simulink model "Sistema_4_2024b"  (R2024b)
settings: Solver=ode15s  StartTime=0.0  StopTime=10  MaxStep=1E-2  RelTol=1e-3
libraries: fl_lib x14, nesl_utility x6, slpidlib x1
settings Model: LastModifiedBy=Ernesto
settings DataIOCC: SaveFormat=Array  SaveOutput=off  SignalLogging=off  DSMLogging=off  ReturnWorkspaceOutputs=off  TimeSaveName=t
settings DebuggingCC: AlgebraicLoopMsg=none  ArtificialAlgebraicLoopMsg=none  MaxConsecutiveZCsMsg=none
settings ModelReferenceCC: UpdateModelReferenceTargets=IfOutOfDate
settings RTWCC: GPUComputeCapability=7.5
settings ConfigComp: CovMetricSettings=de  CovBoundaryAbsTol=1.0e-5
settings SimscapeCC: SimscapeNominalValues="[{\"value\":\"1\",\"unit\":\"A\"},{\"value\":\"1\",\"unit\":\"bar\"},{\"value\":\"1\",\"unit\":\"cm^2\"},{\"value\":\"1\",\"unit\":\"cm^3/s\"},{\"value\":\"1\",\"unit\":\"kJ/kg\"},{\"value\":\"1\",\"unit\":\"kW\"},{\"value\":\"1\",\"unit\":\"l\"},{\"value\":\"1\",\"unit\":\"N\"},{\"value\":\"1\",\"unit\":\"N*m\"},{\"value\":\"1\",\"unit\":\"V\"},{\"value\":\"0.001\",\"unit\":\"Wb\"}]"  SimscapeLogType=all  SimscapeLogDataHistory=10000  SimscapeUseEnergyAccounting=off

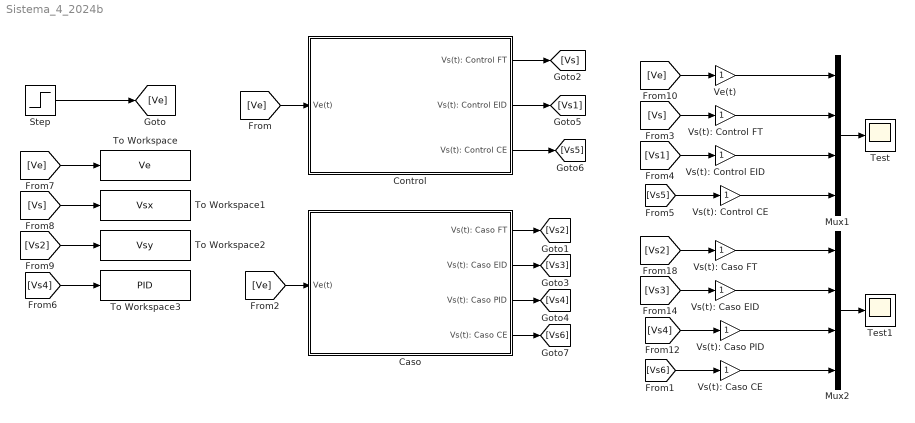
== system Sistema_4_2024b ==
  " Ve(t)" : Gain
  " Vs(t): Caso CE" : Gain
  " Vs(t): Caso EID" : Gain
  " Vs(t): Caso FT" : Gain
  " Vs(t): Caso PID" : Gain
  " Vs(t): Control CE" : Gain
  " Vs(t): Control EID" : Gain
  " Vs(t): Control FT" : Gain
  Caso : Subsystem
  Control : Subsystem
  Mux1 : Mux
  Mux2 : Mux
  Step : Step  Time=0  SampleTime=0
  Test : Scope
  Test1 : Scope
  To Workspace : ToWorkspace  VariableName=Ve  SampleTime=-1
  To Workspace1 : ToWorkspace  VariableName=Vsx  SampleTime=-1
  To Workspace2 : ToWorkspace  VariableName=Vsy  SampleTime=-1
  To Workspace3 : ToWorkspace  VariableName=PID  SampleTime=-1
  wires:
  [Ve] -> Control/1(Ve(t))
  Control/1(Vs(t): Control FT) -> [Vs]
  [Ve] -> Caso/1(Ve(t))
  Caso/1(Vs(t): Caso FT) -> [Vs2]
  Mux1/1 -> Test/1
  [Vs] -> " Vs(t): Control FT"/1
  [Vs1] -> " Vs(t): Control EID"/1
  Step/1 -> [Ve]
  Caso/2(Vs(t): Caso EID) -> [Vs3]
  [Ve] -> " Ve(t)"/1
  " Vs(t): Control FT"/1 -> Mux1/2
  " Ve(t)"/1 -> Mux1/1
  " Vs(t): Control EID"/1 -> Mux1/3
  Control/2(Vs(t): Control EID) -> [Vs1]
  [Ve] -> To Workspace/1
  [Vs] -> To Workspace1/1
  [Vs2] -> To Workspace2/1
  Caso/3(Vs(t): Caso PID) -> [Vs4]
  Control/3(Vs(t): Control CE) -> [Vs5]
  [Vs5] -> " Vs(t): Control CE"/1
  [Vs4] -> " Vs(t): Caso PID"/1
  [Vs3] -> " Vs(t): Caso EID"/1
  [Vs2] -> " Vs(t): Caso FT"/1
  Mux2/1 -> Test1/1
  " Vs(t): Control CE"/1 -> Mux1/4
  Caso/4(Vs(t): Caso CE) -> [Vs6]
  [Vs6] -> " Vs(t): Caso CE"/1
  " Vs(t): Caso FT"/1 -> Mux2/1
  " Vs(t): Caso EID"/1 -> Mux2/2
  " Vs(t): Caso PID"/1 -> Mux2/3
  " Vs(t): Caso CE"/1 -> Mux2/4
  [Vs4] -> To Workspace3/1

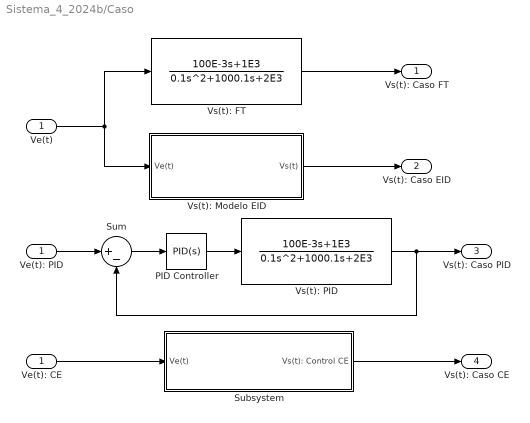
== system Sistema_4_2024b/Caso ==
  Ve(t) : Inport
  PID Controller : slpidlib/PID Controller  Controller=PID  Form=Parallel  TimeDomain=Continuous-time  UseExternalTs=off  SampleTime=-1  IntegratorMethod=Forward Euler  FilterMethod=Forward Euler  ControllerParametersSource=internal  P=13209.9564  I=32316525.9285  UseKiTs=off  D=0.18118  UseExternalDerivativeSource=off  N=521.395873847586  UseFilter=on  TunerSelectOption=Transfer Function Based (PID Tuner App)  InitialConditionSource=internal  InitialConditionForIntegrator=0  InitialConditionForFilter=0  DifferentiatorICPrevScaledInput=0  ExternalReset=none  TrackingMode=off  Kt=1  LimitOutput=off  SatLimitsSource=internal  UpperSaturationLimit=inf  LowerSaturationLimit=-inf  LinearizeAsGain=on  AntiWindupMode=none  Kb=1  LimitIntegrator=off  UpperIntegratorSaturationLimit=inf  LowerIntegratorSaturationLimit=-inf  POutMin=[]  POutMax=[]  IOutMin=[]  IOutMax=[]  DOutMin=[]  DOutMax=[]  NOutMin=[]  NOutMax=[]  SumOutMin=[]  SumOutMax=[]  SaturationOutMin=[]  SaturationOutMax=[]  PParamMin=[]  PParamMax=[]  IParamMin=[]  IParamMax=[]  DParamMin=[]  DParamMax=[]  NParamMin=[]  NParamMax=[]  KbParamMin=[]  KbParamMax=[]  KtParamMin=[]  KtParamMax=[]  KbOutMin=[]  KbOutMax=[]  KtOutMin=[]  KtOutMax=[]  IntegratorOutMin=[]  IntegratorOutMax=[]  FilterOutMin=[]  FilterOutMax=[]  SumI1OutMin=[]  SumI1OutMax=[]  SumI2OutMin=[]  SumI2OutMax=[]  SumI3OutMin=[]  SumI3OutMax=[]  SumI4OutMin=[]  SumI4OutMax=[]  SumDOutMin=[]  SumDOutMax=[]  DifferentiatorOutMin=[]  DifferentiatorOutMax=[]  FilterDiffOutCoefMin=[]  FilterDiffOutCoefMax=[]  ReciprocalOutMin=[]  ReciprocalOutMax=[]  SumDenOutMin=[]  SumDenOutMax=[]  SumNumOutMin=[]  SumNumOutMax=[]  DivideOutMin=[]  DivideOutMax=[]  UdiffTsProdOutMin=[]  UdiffTsProdOutMax=[]  NTsProdOutMin=[]  NTsProdOutMax=[]  UintegralTsProdOutMin=[]  UintegralTsProdOutMax=[]  UngainTsProdOutMin=[]  UngainTsProdOutMax=[]  ClampingZeroOutDataTypeStr=Inherit: Inherit via back propagation  ClampingZeroOutMin=[]  ClampingZeroOutMax=[]  FilterDenConstantOutDataTypeStr=Inherit: Inherit via back propagation  FilterDenConstantOutMin=[]  FilterDenConstantOutMax=[]  PCopyOutDataTypeStr=Inherit: Inherit via back propagation  PCopyOutMin=[]  PCopyOutMax=[]  NCopyOutDataTypeStr=Inherit: Inherit via back propagation  NCopyOutMin=[]  NCopyOutMax=[]  IntegratorContinuousStateAttributes=''  IntegratorStateMustResolveToSignalObject=off  IntegratorRTWStateStorageClass=Auto  FilterContinuousStateAttributes=''  FilterStateMustResolveToSignalObject=off  FilterRTWStateStorageClass=Auto  ParallelPVariant=InternalParameters  IdealPVariant=Disabled  IVariant=InternalParameters  DVariant=InternalParameters  IntegratorVariant=Continuous  SatVariant=Disabled  AWVariant=Passthrough  PCopyVariant=Disabled  TRVariant=Disabled  FdbkBlocksVariant=Forward  IdealPFdbkVariant=Disabled  SatFdbkVariant=Disabled  DerivativeFilterVariant=ContFilter  NVariant=InternalParameters  NCopyVariant=Disabled  FilterICVariant=InternalICsFilter  IntegratorICVariant=InternalICs  ExternalResetVariant=Disabled  TRSumVariant=Passthrough  SumFdbkVariant=Disabled  SumVariant=Sum_PID  TsampFilterVariant=InternalTs  TsampNgainVariant=Passthrough  TsampIntegralVariant=Disabled_SignalSpec  ExternalSaturationOutDataTypeStr=Inherit: Same as second input  DerivativeSourceVariant=ErrorSignal  PreIntVariant=InternalPreInt
  Subsystem : Subsystem
  Sum : Sum  Inputs=|+-
  Ve(t): CE : InportShadow
  Ve(t): PID : InportShadow
  Vs(t): FT : TransferFcn  Numerator=[100E-3, 1E3]  Denominator=[0.1, 1000.1, 2E3]
  Vs(t): Modelo EID : Subsystem
  Vs(t): PID : TransferFcn  Numerator=[100E-3, 1E3]  Denominator=[0.1, 1000.1, 2E3]
  Vs(t): Caso FT : Outport
  Vs(t): Caso EID : Outport  Port=2
  Vs(t): Caso PID : Outport  Port=3
  Vs(t): Caso CE : Outport  Port=4
  wires:
  Ve(t)/1 -> Vs(t): Modelo EID/1(Ve(t)), Vs(t): FT/1
  Vs(t): FT/1 -> Vs(t): Caso FT/1
  Vs(t): Modelo EID/1(Vs(t)) -> Vs(t): Caso EID/1
  PID Controller/1 -> Vs(t): PID/1
  Sum/1 -> PID Controller/1
  Ve(t): PID/1 -> Sum/1
  Vs(t): PID/1 -> Sum/2, Vs(t): Caso PID/1
  Ve(t): CE/1 -> Subsystem/1(Ve(t))
  Subsystem/1(Vs(t): Control CE) -> Vs(t): Caso CE/1

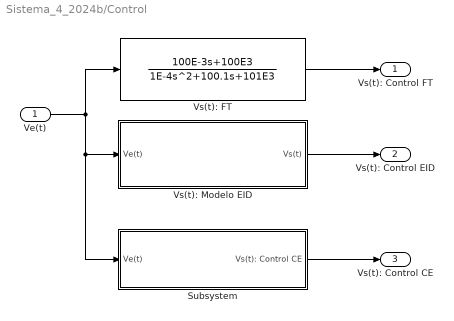
== system Sistema_4_2024b/Control ==
  Ve(t) : Inport
  Subsystem : Subsystem
  Vs(t): FT : TransferFcn  Numerator=[100E-3, 100E3]  Denominator=[1E-4, 100.1, 101E3]
  Vs(t): Modelo EID : Subsystem
  Vs(t): Control FT : Outport
  Vs(t): Control EID : Outport  Port=2
  Vs(t): Control CE : Outport  Port=3
  wires:
  Ve(t)/1 -> Subsystem/1(Ve(t)), Vs(t): Modelo EID/1(Ve(t)), Vs(t): FT/1
  Vs(t): FT/1 -> Vs(t): Control FT/1
  Vs(t): Modelo EID/1(Vs(t)) -> Vs(t): Control EID/1
  Subsystem/1(Vs(t): Control CE) -> Vs(t): Control CE/1

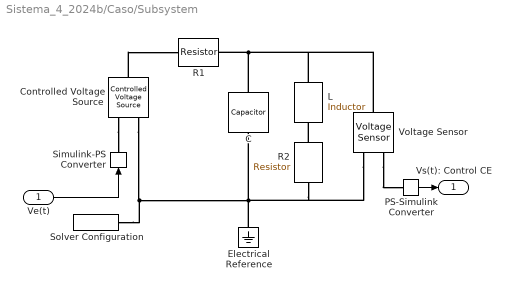
== system Sistema_4_2024b/Caso/Subsystem ==
  Ve(t) : Inport
  C : fl_lib/Electrical/Electrical Elements/Capacitor  c=1000 uF  r=1e-6 Ohm  g=0 1/Ohm  i_specify=off  i_priority=None  i=0 A  i_nominal_specify=off  i_nominal_value=1  i_nominal_unit=A  v_specify=off  v_priority=None  v=0 V  v_nominal_specify=off  v_nominal_value=1  v_nominal_unit=V  vc_specify=off  vc_priority=High  vc=0 V  vc_nominal_specify=off  vc_nominal_value=1  vc_nominal_unit=V
  Controlled Voltage Source : fl_lib/Electrical/Electrical Sources/Controlled Voltage Source
  Electrical Reference : fl_lib/Electrical/Electrical Elements/Electrical Reference
  L : fl_lib/Electrical/Electrical Elements/Inductor  l=100 mH  r=0 Ohm  g=1e-9 1/Ohm  i_specify=off  i_priority=None  i=0 A  i_nominal_specify=off  i_nominal_value=1  i_nominal_unit=A  v_specify=off  v_priority=None  v=0 V  v_nominal_specify=off  v_nominal_value=1  v_nominal_unit=V  i_L_specify=off  i_L_priority=High  i_L=0 A  i_L_nominal_specify=off  i_L_nominal_value=1  i_L_nominal_unit=A
  PS-Simulink Converter : nesl_utility/PS-Simulink Converter  PhysicalDomain=network_engine_domain  SubClassName=ps_output  LeftPortType=input  RightPortType=output  PseudoPeriodic=off  Frequencies=[]  VectorFormat=inherit  Unit=inherit  AffineConversion=off
  R1 : fl_lib/Electrical/Electrical Elements/Resistor  R=1 kOhm  i_specify=off  i_priority=None  i=0 A  i_nominal_specify=off  i_nominal_value=1  i_nominal_unit=A  v_specify=off  v_priority=None  v=0 V  v_nominal_specify=off  v_nominal_value=1  v_nominal_unit=V
  R2 : fl_lib/Electrical/Electrical Elements/Resistor  R=1 kOhm  i_specify=off  i_priority=None  i=0 A  i_nominal_specify=off  i_nominal_value=1  i_nominal_unit=A  v_specify=off  v_priority=None  v=0 V  v_nominal_specify=off  v_nominal_value=1  v_nominal_unit=V
  Simulink-PS Converter : nesl_utility/Simulink-PS Converter  PhysicalDomain=network_engine_domain  SubClassName=ps_input  LeftPortType=input  RightPortType=output  PseudoPeriodic=off  Frequencies=[]  NoiseDistribution=none  NoiseParameters=[]  Unit=1  AffineConversion=off  FilteringAndDerivatives=provide  SimscapeFilterOrder=1  InputFilterTimeConstant=0.001  UdotUserProvided=0
  Solver Configuration : nesl_utility/Solver Configuration  PhysicalDomain=network_engine_domain  SubClassName=solver  LeftPortType=input  RightPortType=generic  Tones=[]  Harmonics=[]  SimulateNoise=off  Profile=off  UseLocalSampling=off  EnableSwitchedLinearOptims=on  FrequencyDomain=off  UseCCode=off  RelTol=0.001  AbsTol=0.001  MinStep=1e-09  ToWorkspace=off  RevertToSquareIcSolve=off  NumHomotopyIterations=100  PhasorMode=off  PhasorModeNumHarmonics=1  ConsistencySolver=NEWTON_XTOL_AFTER_FTOL  CanonicalOrdering=CANONICAL  OptimizeIntermediates=OPTIMIZED  MulticoreSolverChoice=BACKWARD_EULER  IndexReductionMethod=DerivativeReplacement  DoDC=off  ResidualTolerance=1e-09  ConsistencyTolSource=GLOBAL  ConsistencyAbsTol=0.001  ConsistencyRelTol=0.001  ConsistencyTolFactor=0.001  UseLocalSolver=off  LocalSolverChoice=NE_BACKWARD_EULER_ADVANCER  ResolveIndetEquations=on  FunctionEvalNumThread=1  LocalSolverSampleTime=0.001  DoFixedCost=off  MaxNonlinIter=3  MaxModeIter=2  ComputeImpulses=off  ImpulseIterations=2  LinearAlgebra=auto  LinearAlgebraNumThread=0  EquationFormulation=NE_TIME_EF  DelaysMemoryBudget=1024  AutomaticFiltering=on  FilteringTimeConstant=0.001  PartitionStorageMethod=AS_NEEDED  PartitionMemoryBudget=1024  PartitionMethod=BALANCED  MultibodyUseLocalSolver=off  MultibodyLocalSolverChoice=ODE1  MultibodyLocalSolverSampleTime=0.001
  Voltage Sensor : fl_lib/Electrical/Electrical Sensors/Voltage Sensor
  Vs(t): Control CE : Outport
  wires:
  Ve(t)/1 -> Simulink-PS Converter/1
  PS-Simulink Converter/1 -> Vs(t): Control CE/1
  connections:
  Controlled Voltage Source/RConn1 -- Simulink-PS Converter/RConn1
  Controlled Voltage Source/LConn1 -- R1/LConn1
  C/LConn1 -- R1/RConn1 -- L/LConn1 -- Voltage Sensor/LConn1
  Solver Configuration/RConn1 -- Controlled Voltage Source/RConn2 -- C/RConn1 -- Electrical Reference/LConn1 -- R2/RConn1 -- Voltage Sensor/RConn2
  R2/LConn1 -- L/RConn1
  Voltage Sensor/RConn1 -- PS-Simulink Converter/LConn1

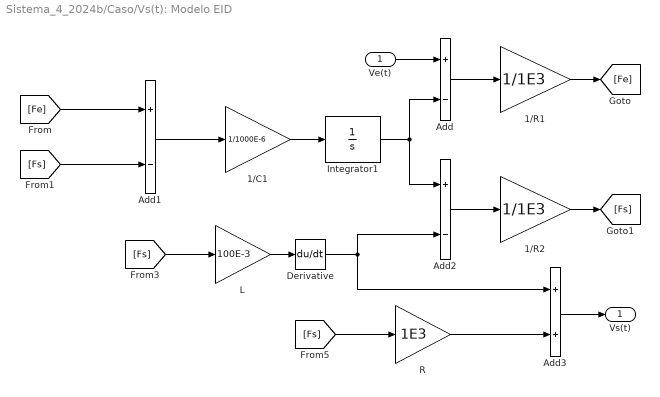
== system Sistema_4_2024b/Caso/Vs(t): Modelo EID ==
  Ve(t) : Inport
  1/C1 : Gain  Gain=1/1000E-6
  1/R1 : Gain  Gain=1/1E3
  1/R2 : Gain  Gain=1/1E3
  Add : Sum  Inputs=+-
  Add1 : Sum  Inputs=+-
  Add2 : Sum  Inputs=+-
  Add3 : Sum
  Derivative : Derivative
  Integrator1 : Integrator
  L : Gain  Gain=100E-3
  R : Gain  Gain=1E3
  Vs(t) : Outport
  wires:
  1/R1/1 -> [Fe]
  [Fs] -> Add1/2
  [Fe] -> Add1/1
  [Fs] -> L/1
  Add/1 -> 1/R1/1
  [Fs] -> R/1
  1/C1/1 -> Integrator1/1
  Ve(t)/1 -> Add/1
  Add1/1 -> 1/C1/1
  Add2/1 -> 1/R2/1
  1/R2/1 -> [Fs]
  Add3/1 -> Vs(t)/1
  Integrator1/1 -> Add2/1, Add/2
  R/1 -> Add3/2
  L/1 -> Derivative/1
  Derivative/1 -> Add3/1, Add2/2

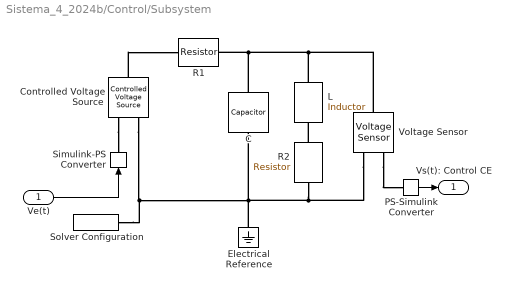
== system Sistema_4_2024b/Control/Subsystem ==
  Ve(t) : Inport
  C : fl_lib/Electrical/Electrical Elements/Capacitor  c=1 uF  r=1e-6 Ohm  g=0 1/Ohm  i_specify=off  i_priority=None  i=0 A  i_nominal_specify=off  i_nominal_value=1  i_nominal_unit=A  v_specify=off  v_priority=None  v=0 V  v_nominal_specify=off  v_nominal_value=1  v_nominal_unit=V  vc_specify=off  vc_priority=High  vc=0 V  vc_nominal_specify=off  vc_nominal_value=1  vc_nominal_unit=V
  Controlled Voltage Source : fl_lib/Electrical/Electrical Sources/Controlled Voltage Source
  Electrical Reference : fl_lib/Electrical/Electrical Elements/Electrical Reference
  L : fl_lib/Electrical/Electrical Elements/Inductor  l=100 mH  r=0 Ohm  g=1e-9 1/Ohm  i_specify=off  i_priority=None  i=0 A  i_nominal_specify=off  i_nominal_value=1  i_nominal_unit=A  v_specify=off  v_priority=None  v=0 V  v_nominal_specify=off  v_nominal_value=1  v_nominal_unit=V  i_L_specify=off  i_L_priority=High  i_L=0 A  i_L_nominal_specify=off  i_L_nominal_value=1  i_L_nominal_unit=A
  PS-Simulink Converter : nesl_utility/PS-Simulink Converter  PhysicalDomain=network_engine_domain  SubClassName=ps_output  LeftPortType=input  RightPortType=output  PseudoPeriodic=off  Frequencies=[]  VectorFormat=inherit  Unit=inherit  AffineConversion=off
  R1 : fl_lib/Electrical/Electrical Elements/Resistor  R=1 kOhm  i_specify=off  i_priority=None  i=0 A  i_nominal_specify=off  i_nominal_value=1  i_nominal_unit=A  v_specify=off  v_priority=None  v=0 V  v_nominal_specify=off  v_nominal_value=1  v_nominal_unit=V
  R2 : fl_lib/Electrical/Electrical Elements/Resistor  R=100 kOhm  i_specify=off  i_priority=None  i=0 A  i_nominal_specify=off  i_nominal_value=1  i_nominal_unit=A  v_specify=off  v_priority=None  v=0 V  v_nominal_specify=off  v_nominal_value=1  v_nominal_unit=V
  Simulink-PS Converter : nesl_utility/Simulink-PS Converter  PhysicalDomain=network_engine_domain  SubClassName=ps_input  LeftPortType=input  RightPortType=output  PseudoPeriodic=off  Frequencies=[]  NoiseDistribution=none  NoiseParameters=[]  Unit=1  AffineConversion=off  FilteringAndDerivatives=provide  SimscapeFilterOrder=1  InputFilterTimeConstant=0.001  UdotUserProvided=0
  Solver Configuration : nesl_utility/Solver Configuration  PhysicalDomain=network_engine_domain  SubClassName=solver  LeftPortType=input  RightPortType=generic  Tones=[]  Harmonics=[]  SimulateNoise=off  Profile=off  UseLocalSampling=off  EnableSwitchedLinearOptims=on  FrequencyDomain=off  UseCCode=off  RelTol=0.001  AbsTol=0.001  MinStep=1e-09  ToWorkspace=off  RevertToSquareIcSolve=off  NumHomotopyIterations=100  PhasorMode=off  PhasorModeNumHarmonics=1  ConsistencySolver=NEWTON_XTOL_AFTER_FTOL  CanonicalOrdering=CANONICAL  OptimizeIntermediates=OPTIMIZED  MulticoreSolverChoice=BACKWARD_EULER  IndexReductionMethod=DerivativeReplacement  DoDC=off  ResidualTolerance=1e-09  ConsistencyTolSource=GLOBAL  ConsistencyAbsTol=0.001  ConsistencyRelTol=0.001  ConsistencyTolFactor=0.001  UseLocalSolver=off  LocalSolverChoice=NE_BACKWARD_EULER_ADVANCER  ResolveIndetEquations=on  FunctionEvalNumThread=1  LocalSolverSampleTime=0.001  DoFixedCost=off  MaxNonlinIter=3  MaxModeIter=2  ComputeImpulses=off  ImpulseIterations=2  LinearAlgebra=auto  LinearAlgebraNumThread=0  EquationFormulation=NE_TIME_EF  DelaysMemoryBudget=1024  AutomaticFiltering=on  FilteringTimeConstant=0.001  PartitionStorageMethod=AS_NEEDED  PartitionMemoryBudget=1024  PartitionMethod=BALANCED  MultibodyUseLocalSolver=off  MultibodyLocalSolverChoice=ODE1  MultibodyLocalSolverSampleTime=0.001
  Voltage Sensor : fl_lib/Electrical/Electrical Sensors/Voltage Sensor
  Vs(t): Control CE : Outport
  wires:
  Ve(t)/1 -> Simulink-PS Converter/1
  PS-Simulink Converter/1 -> Vs(t): Control CE/1
  connections:
  Controlled Voltage Source/RConn1 -- Simulink-PS Converter/RConn1
  Controlled Voltage Source/LConn1 -- R1/LConn1
  C/LConn1 -- Voltage Sensor/LConn1 -- L/LConn1 -- R1/RConn1
  Electrical Reference/LConn1 -- Voltage Sensor/RConn2 -- R2/RConn1 -- Solver Configuration/RConn1 -- Controlled Voltage Source/RConn2 -- C/RConn1
  R2/LConn1 -- L/RConn1
  Voltage Sensor/RConn1 -- PS-Simulink Converter/LConn1

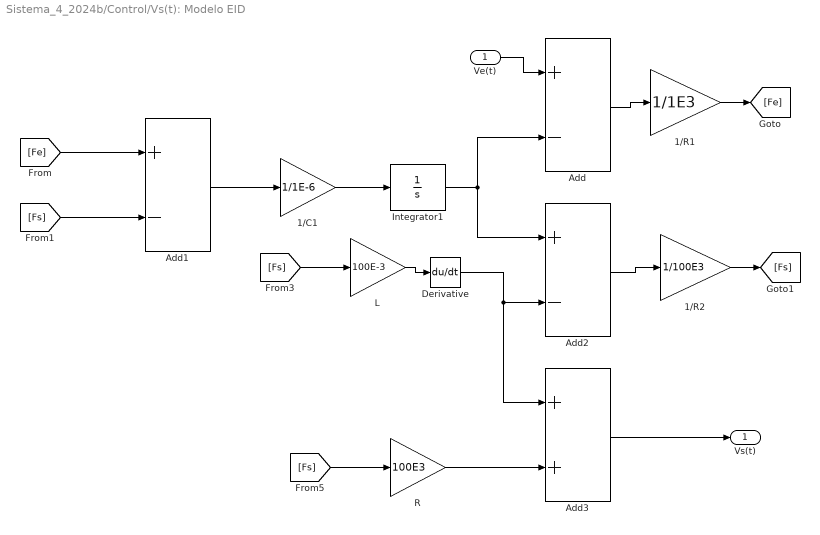
== system Sistema_4_2024b/Control/Vs(t): Modelo EID ==
  Ve(t) : Inport
  1/C1 : Gain  Gain=1/1E-6
  1/R1 : Gain  Gain=1/1E3
  1/R2 : Gain  Gain=1/100E3
  Add : Sum  Inputs=+-
  Add1 : Sum  Inputs=+-
  Add2 : Sum  Inputs=+-
  Add3 : Sum
  Derivative : Derivative
  Integrator1 : Integrator
  L : Gain  Gain=100E-3
  R : Gain  Gain=100E3
  Vs(t) : Outport
  wires:
  1/R1/1 -> [Fe]
  [Fs] -> Add1/2
  [Fe] -> Add1/1
  [Fs] -> L/1
  Add/1 -> 1/R1/1
  [Fs] -> R/1
  1/C1/1 -> Integrator1/1
  Ve(t)/1 -> Add/1
  Add1/1 -> 1/C1/1
  Add2/1 -> 1/R2/1
  1/R2/1 -> [Fs]
  Add3/1 -> Vs(t)/1
  Integrator1/1 -> Add2/1, Add/2
  R/1 -> Add3/2
  L/1 -> Derivative/1
  Derivative/1 -> Add3/1, Add2/2
